simulink model "ads5296x4"  (R2019a)
settings: Solver=VariableStepAuto  StartTime=0.0  StopTime=10.0  RelTol=1e-3
libraries: xbsIndex_r4 x35
settings Model: Creator=qwerty40  LastModifiedBy=jackh
settings DataIOCC: ReturnWorkspaceOutputs=off
settings DebuggingCC: PregeneratedLibrarySubsystemCodeDiagnostic=none  ArithmeticOperatorsInVariantConditions=warning
settings SFSimCC: SimUseLocalCustomCode=off
settings RTWCC: RTWUseLocalCustomCode=off
settings CodeAppCC: StateflowObjectComments=on

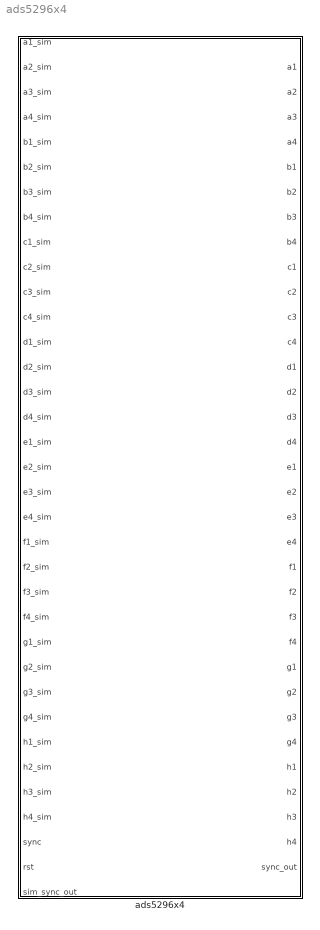
== system ads5296x4 ==
  ads5296x4 : Subsystem  Tag=xps:ads5296x4  mask(ADS5296x4){board_count=2, sample_rate=200, port=0, clockport=0, version=1}
      mask prompts: board_count "Number of quad-chip ADC Boards"; sample_rate "Sample Rate"; port "Which FMC port?"; clockport "Use clock from which FMC board?"; version "Which ADC board version?"
      mask help: 16-input ADC based on the TI ADS5296 chip.
      mask init:
      | % Only board_count is needed by init function
      | ads5296x4_init(gcb, ...
      |     'board_count', board_count);
      mask TypeOptions board_count: 1 | 2 | 3 | 4

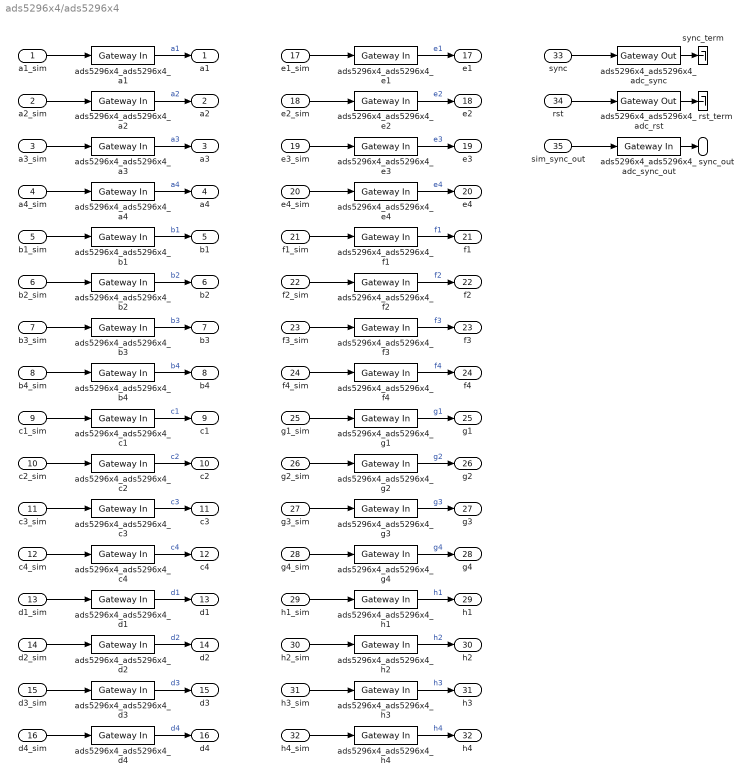
== system ads5296x4/ads5296x4 ==
  a1_sim : Inport
  a2_sim : Inport  Port=2
  a3_sim : Inport  Port=3
  a4_sim : Inport  Port=4
  b1_sim : Inport  Port=5
  b2_sim : Inport  Port=6
  b3_sim : Inport  Port=7
  b4_sim : Inport  Port=8
  c1_sim : Inport  Port=9
  c2_sim : Inport  Port=10
  c3_sim : Inport  Port=11
  c4_sim : Inport  Port=12
  d1_sim : Inport  Port=13
  d2_sim : Inport  Port=14
  d3_sim : Inport  Port=15
  d4_sim : Inport  Port=16
  e1_sim : Inport  Port=17
  e2_sim : Inport  Port=18
  e3_sim : Inport  Port=19
  e4_sim : Inport  Port=20
  f1_sim : Inport  Port=21
  f2_sim : Inport  Port=22
  f3_sim : Inport  Port=23
  f4_sim : Inport  Port=24
  g1_sim : Inport  Port=25
  g2_sim : Inport  Port=26
  g3_sim : Inport  Port=27
  g4_sim : Inport  Port=28
  h1_sim : Inport  Port=29
  h2_sim : Inport  Port=30
  h3_sim : Inport  Port=31
  h4_sim : Inport  Port=32
  sync : Inport  Port=33
  rst : Inport  Port=34
  sim_sync_out : Inport  Port=35
  ads5296x4_ads5296x4_a{1..4} (4 alike) : xbsIndex_r4/Gateway In  gui_display_data_type=Fixed-point  arith_type="Signed  (2's comp)"  n_bits=10  bin_pt=9  preci_type=Single  exp_width=8  frac_width=24  rows=1  columns=1  quantization="Round  (unbiased: +/- Inf)"  overflow=Saturate  period=1  UseAsADC=off  ADCChannel='1'  interface=None  automatic_assignment=on  address_offset=hex2dec('00')  intf_name=''  intf_description=''  default_value=0  timing_constraint=None  locs_specified=off  LOCs={}  io_standard={}  inherit_from_input=off  hdl_port=on  dbl_ovrd=off  block_type=gatewayin
  ads5296x4_ads5296x4_adc_rst : xbsIndex_r4/Gateway Out  inherit_from_input=off  hdl_port=on  rows=1  columns=1  UseAsDAC=off  DACChannel='1'  interface=None  automatic_assignment=on  address_offset=hex2dec('00')  intf_name=''  intf_description=''  timing_constraint=None  locs_specified=off  LOCs={}  io_standard={}  block_type=gatewayout
  ads5296x4_ads5296x4_adc_sync : xbsIndex_r4/Gateway Out  inherit_from_input=off  hdl_port=on  rows=1  columns=1  UseAsDAC=off  DACChannel='1'  interface=None  automatic_assignment=on  address_offset=hex2dec('00')  intf_name=''  intf_description=''  timing_constraint=None  locs_specified=off  LOCs={}  io_standard={}  block_type=gatewayout
  ads5296x4_ads5296x4_adc_sync_out : xbsIndex_r4/Gateway In  gui_display_data_type=Fixed-point  arith_type=Boolean  n_bits=16  bin_pt=14  preci_type=Single  exp_width=8  frac_width=24  rows=1  columns=1  quantization="Round  (unbiased: +/- Inf)"  overflow=Saturate  period=1  UseAsADC=off  ADCChannel='1'  interface=None  automatic_assignment=on  address_offset=hex2dec('00')  intf_name=''  intf_description=''  default_value=0  timing_constraint=None  locs_specified=off  LOCs={}  io_standard={}  inherit_from_input=off  hdl_port=on  dbl_ovrd=off  block_type=gatewayin
  ads5296x4_ads5296x4_b{1..4} (4 alike) : xbsIndex_r4/Gateway In  gui_display_data_type=Fixed-point  arith_type="Signed  (2's comp)"  n_bits=10  bin_pt=9  preci_type=Single  exp_width=8  frac_width=24  rows=1  columns=1  quantization="Round  (unbiased: +/- Inf)"  overflow=Saturate  period=1  UseAsADC=off  ADCChannel='1'  interface=None  automatic_assignment=on  address_offset=hex2dec('00')  intf_name=''  intf_description=''  default_value=0  timing_constraint=None  locs_specified=off  LOCs={}  io_standard={}  inherit_from_input=off  hdl_port=on  dbl_ovrd=off  block_type=gatewayin
  ads5296x4_ads5296x4_c{1..4} (4 alike) : xbsIndex_r4/Gateway In  gui_display_data_type=Fixed-point  arith_type="Signed  (2's comp)"  n_bits=10  bin_pt=9  preci_type=Single  exp_width=8  frac_width=24  rows=1  columns=1  quantization="Round  (unbiased: +/- Inf)"  overflow=Saturate  period=1  UseAsADC=off  ADCChannel='1'  interface=None  automatic_assignment=on  address_offset=hex2dec('00')  intf_name=''  intf_description=''  default_value=0  timing_constraint=None  locs_specified=off  LOCs={}  io_standard={}  inherit_from_input=off  hdl_port=on  dbl_ovrd=off  block_type=gatewayin
  ads5296x4_ads5296x4_d{1..4} (4 alike) : xbsIndex_r4/Gateway In  gui_display_data_type=Fixed-point  arith_type="Signed  (2's comp)"  n_bits=10  bin_pt=9  preci_type=Single  exp_width=8  frac_width=24  rows=1  columns=1  quantization="Round  (unbiased: +/- Inf)"  overflow=Saturate  period=1  UseAsADC=off  ADCChannel='1'  interface=None  automatic_assignment=on  address_offset=hex2dec('00')  intf_name=''  intf_description=''  default_value=0  timing_constraint=None  locs_specified=off  LOCs={}  io_standard={}  inherit_from_input=off  hdl_port=on  dbl_ovrd=off  block_type=gatewayin
  ads5296x4_ads5296x4_e{1..4} (4 alike) : xbsIndex_r4/Gateway In  gui_display_data_type=Fixed-point  arith_type="Signed  (2's comp)"  n_bits=10  bin_pt=9  preci_type=Single  exp_width=8  frac_width=24  rows=1  columns=1  quantization="Round  (unbiased: +/- Inf)"  overflow=Saturate  period=1  UseAsADC=off  ADCChannel='1'  interface=None  automatic_assignment=on  address_offset=hex2dec('00')  intf_name=''  intf_description=''  default_value=0  timing_constraint=None  locs_specified=off  LOCs={}  io_standard={}  inherit_from_input=off  hdl_port=on  dbl_ovrd=off  block_type=gatewayin
  ads5296x4_ads5296x4_f{1..4} (4 alike) : xbsIndex_r4/Gateway In  gui_display_data_type=Fixed-point  arith_type="Signed  (2's comp)"  n_bits=10  bin_pt=9  preci_type=Single  exp_width=8  frac_width=24  rows=1  columns=1  quantization="Round  (unbiased: +/- Inf)"  overflow=Saturate  period=1  UseAsADC=off  ADCChannel='1'  interface=None  automatic_assignment=on  address_offset=hex2dec('00')  intf_name=''  intf_description=''  default_value=0  timing_constraint=None  locs_specified=off  LOCs={}  io_standard={}  inherit_from_input=off  hdl_port=on  dbl_ovrd=off  block_type=gatewayin
  ads5296x4_ads5296x4_g{1..4} (4 alike) : xbsIndex_r4/Gateway In  gui_display_data_type=Fixed-point  arith_type="Signed  (2's comp)"  n_bits=10  bin_pt=9  preci_type=Single  exp_width=8  frac_width=24  rows=1  columns=1  quantization="Round  (unbiased: +/- Inf)"  overflow=Saturate  period=1  UseAsADC=off  ADCChannel='1'  interface=None  automatic_assignment=on  address_offset=hex2dec('00')  intf_name=''  intf_description=''  default_value=0  timing_constraint=None  locs_specified=off  LOCs={}  io_standard={}  inherit_from_input=off  hdl_port=on  dbl_ovrd=off  block_type=gatewayin
  ads5296x4_ads5296x4_h{1..4} (4 alike) : xbsIndex_r4/Gateway In  gui_display_data_type=Fixed-point  arith_type="Signed  (2's comp)"  n_bits=10  bin_pt=9  preci_type=Single  exp_width=8  frac_width=24  rows=1  columns=1  quantization="Round  (unbiased: +/- Inf)"  overflow=Saturate  period=1  UseAsADC=off  ADCChannel='1'  interface=None  automatic_assignment=on  address_offset=hex2dec('00')  intf_name=''  intf_description=''  default_value=0  timing_constraint=None  locs_specified=off  LOCs={}  io_standard={}  inherit_from_input=off  hdl_port=on  dbl_ovrd=off  block_type=gatewayin
  rst_term : Terminator
  sync_term : Terminator
  a1 : Outport
  a2 : Outport  Port=2
  a3 : Outport  Port=3
  a4 : Outport  Port=4
  b1 : Outport  Port=5
  b2 : Outport  Port=6
  b3 : Outport  Port=7
  b4 : Outport  Port=8
  c1 : Outport  Port=9
  c2 : Outport  Port=10
  c3 : Outport  Port=11
  c4 : Outport  Port=12
  d1 : Outport  Port=13
  d2 : Outport  Port=14
  d3 : Outport  Port=15
  d4 : Outport  Port=16
  e1 : Outport  Port=17
  e2 : Outport  Port=18
  e3 : Outport  Port=19
  e4 : Outport  Port=20
  f1 : Outport  Port=21
  f2 : Outport  Port=22
  f3 : Outport  Port=23
  f4 : Outport  Port=24
  g1 : Outport  Port=25
  g2 : Outport  Port=26
  g3 : Outport  Port=27
  g4 : Outport  Port=28
  h1 : Outport  Port=29
  h2 : Outport  Port=30
  h3 : Outport  Port=31
  h4 : Outport  Port=32
  sync_out : Outport  Port=33
  wires:
  a1_sim/1 -> ads5296x4_ads5296x4_a1/1
  ads5296x4_ads5296x4_a1/1 -> a1/1  "a1"
  a2_sim/1 -> ads5296x4_ads5296x4_a2/1
  ads5296x4_ads5296x4_a2/1 -> a2/1  "a2"
  a3_sim/1 -> ads5296x4_ads5296x4_a3/1
  ads5296x4_ads5296x4_a3/1 -> a3/1  "a3"
  a4_sim/1 -> ads5296x4_ads5296x4_a4/1
  ads5296x4_ads5296x4_a4/1 -> a4/1  "a4"
  b1_sim/1 -> ads5296x4_ads5296x4_b1/1
  ads5296x4_ads5296x4_b1/1 -> b1/1  "b1"
  b2_sim/1 -> ads5296x4_ads5296x4_b2/1
  ads5296x4_ads5296x4_b2/1 -> b2/1  "b2"
  b3_sim/1 -> ads5296x4_ads5296x4_b3/1
  ads5296x4_ads5296x4_b3/1 -> b3/1  "b3"
  b4_sim/1 -> ads5296x4_ads5296x4_b4/1
  ads5296x4_ads5296x4_b4/1 -> b4/1  "b4"
  c1_sim/1 -> ads5296x4_ads5296x4_c1/1
  ads5296x4_ads5296x4_c1/1 -> c1/1  "c1"
  c2_sim/1 -> ads5296x4_ads5296x4_c2/1
  ads5296x4_ads5296x4_c2/1 -> c2/1  "c2"
  c3_sim/1 -> ads5296x4_ads5296x4_c3/1
  ads5296x4_ads5296x4_c3/1 -> c3/1  "c3"
  c4_sim/1 -> ads5296x4_ads5296x4_c4/1
  ads5296x4_ads5296x4_c4/1 -> c4/1  "c4"
  d1_sim/1 -> ads5296x4_ads5296x4_d1/1
  ads5296x4_ads5296x4_d1/1 -> d1/1  "d1"
  d2_sim/1 -> ads5296x4_ads5296x4_d2/1
  ads5296x4_ads5296x4_d2/1 -> d2/1  "d2"
  d3_sim/1 -> ads5296x4_ads5296x4_d3/1
  ads5296x4_ads5296x4_d3/1 -> d3/1  "d3"
  d4_sim/1 -> ads5296x4_ads5296x4_d4/1
  ads5296x4_ads5296x4_d4/1 -> d4/1  "d4"
  e1_sim/1 -> ads5296x4_ads5296x4_e1/1
  ads5296x4_ads5296x4_e1/1 -> e1/1  "e1"
  e2_sim/1 -> ads5296x4_ads5296x4_e2/1
  ads5296x4_ads5296x4_e2/1 -> e2/1  "e2"
  e3_sim/1 -> ads5296x4_ads5296x4_e3/1
  ads5296x4_ads5296x4_e3/1 -> e3/1  "e3"
  e4_sim/1 -> ads5296x4_ads5296x4_e4/1
  ads5296x4_ads5296x4_e4/1 -> e4/1  "e4"
  f1_sim/1 -> ads5296x4_ads5296x4_f1/1
  ads5296x4_ads5296x4_f1/1 -> f1/1  "f1"
  f2_sim/1 -> ads5296x4_ads5296x4_f2/1
  ads5296x4_ads5296x4_f2/1 -> f2/1  "f2"
  f3_sim/1 -> ads5296x4_ads5296x4_f3/1
  ads5296x4_ads5296x4_f3/1 -> f3/1  "f3"
  f4_sim/1 -> ads5296x4_ads5296x4_f4/1
  ads5296x4_ads5296x4_f4/1 -> f4/1  "f4"
  g1_sim/1 -> ads5296x4_ads5296x4_g1/1
  ads5296x4_ads5296x4_g1/1 -> g1/1  "g1"
  g2_sim/1 -> ads5296x4_ads5296x4_g2/1
  ads5296x4_ads5296x4_g2/1 -> g2/1  "g2"
  g3_sim/1 -> ads5296x4_ads5296x4_g3/1
  ads5296x4_ads5296x4_g3/1 -> g3/1  "g3"
  g4_sim/1 -> ads5296x4_ads5296x4_g4/1
  ads5296x4_ads5296x4_g4/1 -> g4/1  "g4"
  h1_sim/1 -> ads5296x4_ads5296x4_h1/1
  ads5296x4_ads5296x4_h1/1 -> h1/1  "h1"
  h2_sim/1 -> ads5296x4_ads5296x4_h2/1
  ads5296x4_ads5296x4_h2/1 -> h2/1  "h2"
  h3_sim/1 -> ads5296x4_ads5296x4_h3/1
  ads5296x4_ads5296x4_h3/1 -> h3/1  "h3"
  h4_sim/1 -> ads5296x4_ads5296x4_h4/1
  ads5296x4_ads5296x4_h4/1 -> h4/1  "h4"
  sync/1 -> ads5296x4_ads5296x4_adc_sync/1
  ads5296x4_ads5296x4_adc_sync/1 -> sync_term/1
  rst/1 -> ads5296x4_ads5296x4_adc_rst/1
  ads5296x4_ads5296x4_adc_rst/1 -> rst_term/1
  sim_sync_out/1 -> ads5296x4_ads5296x4_adc_sync_out/1
  ads5296x4_ads5296x4_adc_sync_out/1 -> sync_out/1
